simulink model "SimulacionesDT_LUCIA_con_integral"  (R2026b)
settings: Solver=ode15s  StopTime=20
values from neighbouring files (symbols this model uses):
  alpha_Cu = 3.9e-3    (= 0.0039)    [coeficientes.m]
  b_eq = b_m + b_l/(r^2)    (= 2.19444444444e-05)    [coeficientes.m]
  C_ts = 0.818    [coeficientes.m]
  g = 9.80665    [coeficientes.m]
  init_I0 = 0    [coeficientes.m]
  init_Id = 0    [coeficientes.m]
  init_Iq = 0    [coeficientes.m]
  init_theta = 0    [coeficientes.m]
  init_Ts = 20    [coeficientes.m]
  init_w = 0    [coeficientes.m]
  J_eq = J_m + J_l/(r^2)    (= 2.84652777778e-05)    [coeficientes.m]
  k_l = k_l_min + m_l*l_l    (= 0.5)    [coeficientes.m]
  Kd_mov = wn_mov * (2*zeta_mov + 1) * J_eq    (= 0.0569305555556)    [coeficientes.m]
  Ki_mov = wn_mov^3 * J_eq    (= 14574.2222222)    [coeficientes.m]
  Kp_mov = wn_mov^2 * (2*zeta_mov + 1) * J_eq    (= 45.5444444444)    [coeficientes.m]
  L_d = 6.6e-3    (= 0.0066)    [coeficientes.m]
  L_ls = 0.8e-3    (= 0.0008)    [coeficientes.m]
  L_q = 5.8e-3    (= 0.0058)    [coeficientes.m]
  lambda = 0.016    [coeficientes.m]
  Pp = 3    [coeficientes.m]
  r = 120.0    (= 120)    [coeficientes.m]
  R0 = abs(p)*L_ls    [coeficientes.m]
  R_sREF = 1.02    [coeficientes.m]
  R_tsamb = 146.7    [coeficientes.m]
  Rd = abs(p)*L_d    [coeficientes.m]
  Rq = abs(p)*L_q    [coeficientes.m]
  T_sREF = 20    [coeficientes.m]
libraries: eeTransforms x12
(part 2 of 2)

== system SimulacionesDT_LUCIA_con_integral/Sistema con Controlador de Torque Equivalente y sensores ideales1/Modulador de Torque Equivalente/Subsystem ==
  T°s : Inport
  Constant1 : Constant  Value=T_sREF
  Constant2 : Constant
  Gain5 : Gain  Gain=alpha_Cu
  Gain6 : Gain  Gain=R_sREF
  Sum3 : Sum  Inputs=+-|
  Sum4 : Sum  Inputs=|++
  R_s : Outport
  wires:
  Sum3/1 -> Gain5/1
  Sum4/1 -> Gain6/1
  Constant2/1 -> Sum4/2
  Constant1/1 -> Sum3/2
  Gain6/1 -> R_s/1  "R_s"
  Gain5/1 -> Sum4/1
  T°s/1 -> Sum3/1

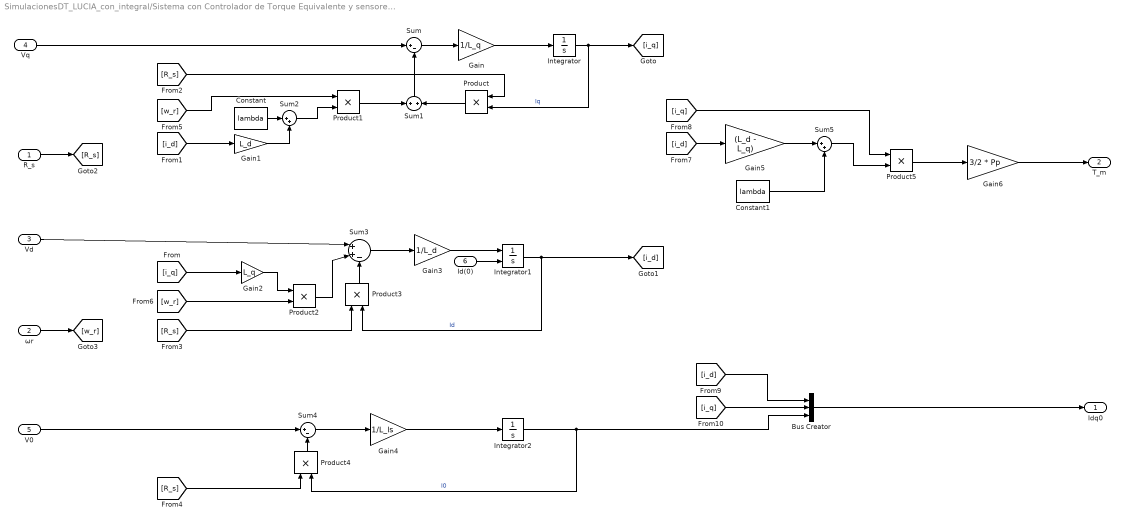
== system SimulacionesDT_LUCIA_con_integral/Sistema con Controlador de Torque Equivalente y sensores ideales1/Planta (Modelo Global No Lineal)/Subsistema Electromagnetico ==
  R_s : Inport
  ωr : Inport  Port=2
  Vd : Inport  Port=3
  Vq : Inport  Port=4
  V0 : Inport  Port=5
  Id(0) : Inport  Port=6
  Bus Creator : BusCreator  Inputs=3
  Constant : Constant  Value=lambda
  Constant1 : Constant  Value=lambda
  Gain : Gain  Gain=1/L_q
  Gain1 : Gain  Gain=L_d
  Gain2 : Gain  Gain=L_q
  Gain3 : Gain  Gain=1/L_d
  Gain4 : Gain  Gain=1/L_ls
  Gain5 : Gain  Gain=(L_d - L_q)
  Gain6 : Gain  Gain=3/2 * Pp
  Integrator : Integrator  InitialCondition=init_Iq
  Integrator1 : Integrator  InitialConditionSource=external  InitialCondition=init_Id
  Integrator2 : Integrator  InitialCondition=init_I0
  Product{,1..5} (6 alike) : Product
  Sum : Sum  Inputs=|+-
  Sum1 : Sum
  Sum2 : Sum  Inputs=|++
  Sum3 : Sum  Inputs=|++-
  Sum4 : Sum  Inputs=|+-
  Sum5 : Sum  Inputs=|++
  Idq0 : Outport
  T_m : Outport  Port=2
  wires:
  [i_q] -> Bus Creator/2
  [i_d] -> Bus Creator/1
  Id(0)/1 -> Integrator1/2
  Bus Creator/1 -> Idq0/1
  [i_q] -> Product5/1
  [i_d] -> Gain5/1
  [w_r] -> Product1/1
  ωr/1 -> [w_r]
  [R_s] -> Product4/1
  [R_s] -> Product3/1
  R_s/1 -> [R_s]
  [i_d] -> Gain1/1
  Gain6/1 -> T_m/1
  Product5/1 -> Gain6/1
  Constant1/1 -> Sum5/2
  Integrator1/1 -> Product3/2, [i_d]  "Id"
  Sum5/1 -> Product5/2
  Gain5/1 -> Sum5/1
  V0/1 -> Sum4/1
  Sum4/1 -> Gain4/1
  Gain4/1 -> Integrator2/1
  Integrator2/1 -> Product4/2, Bus Creator/3  "I0"
  Product4/1 -> Sum4/2
  Vd/1 -> Sum3/1
  Sum3/1 -> Gain3/1
  Gain3/1 -> Integrator1/1
  Product3/1 -> Sum3/3
  Gain/1 -> Integrator/1
  Vq/1 -> Sum/1
  Sum/1 -> Gain/1
  Constant/1 -> Sum2/1
  Sum2/1 -> Product1/2
  Gain1/1 -> Sum2/2
  Product1/1 -> Sum1/1
  Sum1/1 -> Sum/2
  Product/1 -> Sum1/2
  [R_s] -> Product/1
  Integrator/1 -> [i_q], Product/2  "Iq"
  [i_q] -> Gain2/1
  Product2/1 -> Sum3/2
  Gain2/1 -> Product2/1
  [w_r] -> Product2/2

== system SimulacionesDT_LUCIA_con_integral/Sistema con Controlador de Torque Equivalente y sensores ideales1/Planta (Modelo Global No Lineal)/Subsistema Mecanico Equivalente ==
  note: $\theta_m$
  note: $\omega_m$
  note: $\dot{\omega}_m$
  note: $T_{ld}$
  note: $T_m$
  T_m : Inport
  T_ld : Inport  Port=2
  g : Inport  Port=3
  ~θm : Inport  Port=4
  Gain : Gain  Gain=1/r
  Gain1 : Gain  Gain=b_eq
  Gain2 : Gain  Gain=k_l/r
  Gain3 : Gain  Gain=1/J_eq
  Gain4 : Gain  Gain=1/r
  Integrator : Integrator  InitialCondition=init_w
  Integrator1 : Integrator  InitialCondition=init_theta
  Product : Product
  Sin : Trigonometry
  Sum : Sum  Inputs=|+-
  Sum1 : Sum  Inputs=+++
  ωm : Outport
  θm : Outport  Port=2
  wires:
  Integrator1/1 -> Gain4/1, θm/1
  Integrator/1 -> Gain1/1, Integrator1/1, ωm/1
  g/1 -> Product/1
  Product/1 -> Sum1/2
  T_ld/1 -> Gain/1
  Gain4/1 -> Sin/1
  Gain3/1 -> Integrator/1
  Gain1/1 -> Sum1/3
  Sin/1 -> Gain2/1
  Gain/1 -> Sum1/1
  Gain2/1 -> Product/2
  Sum1/1 -> Sum/2
  T_m/1 -> Sum/1
  Sum/1 -> Gain3/1

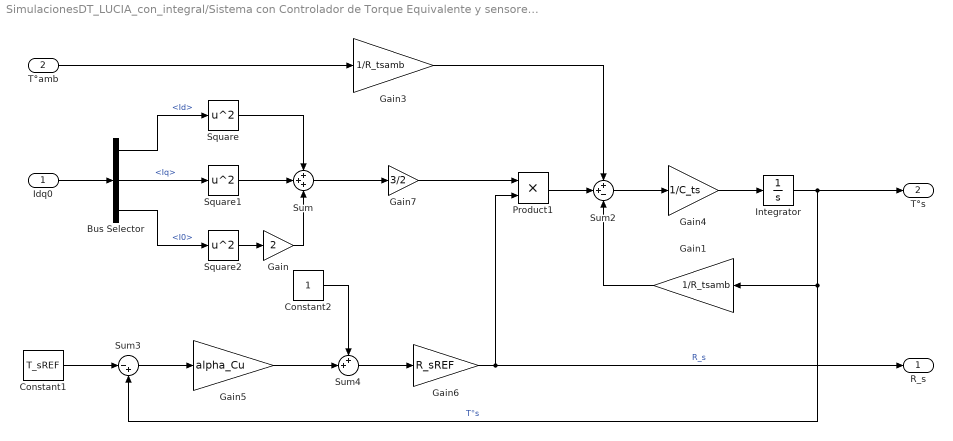
== system SimulacionesDT_LUCIA_con_integral/Sistema con Controlador de Torque Equivalente y sensores ideales1/Planta (Modelo Global No Lineal)/Subsistema Termico ==
  Idq0 : Inport
  T°amb : Inport  Port=2
  Bus Selector : BusSelector  OutputSignals=Id,Iq,I0
  Constant1 : Constant  Value=T_sREF
  Constant2 : Constant
  Gain : Gain  Gain=2
  Gain1 : Gain  Gain=1/R_tsamb
  Gain3 : Gain  Gain=1/R_tsamb
  Gain4 : Gain  Gain=1/C_ts
  Gain5 : Gain  Gain=alpha_Cu
  Gain6 : Gain  Gain=R_sREF
  Gain7 : Gain  Gain=3/2
  Integrator : Integrator  InitialCondition=init_Ts
  Product1 : Product
  Square : Math  Operator=square
  Square1 : Math  Operator=square
  Square2 : Math  Operator=square
  Sum : Sum  Inputs=+++
  Sum2 : Sum  Inputs=++-
  Sum3 : Sum  Inputs=|-+
  Sum4 : Sum  Inputs=++|
  R_s : Outport
  T°s : Outport  Port=2
  wires:
  Bus Selector/3 -> Square2/1  "<I0>"
  Bus Selector/1 -> Square/1  "<Id>"
  Constant2/1 -> Sum4/1
  Idq0/1 -> Bus Selector/1
  Gain3/1 -> Sum2/1
  Gain1/1 -> Sum2/3
  Gain4/1 -> Integrator/1
  Product1/1 -> Sum2/2
  Square/1 -> Sum/1
  Sum2/1 -> Gain4/1
  Square2/1 -> Gain/1
  Sum/1 -> Gain7/1
  T°amb/1 -> Gain3/1
  Sum3/1 -> Gain5/1
  Gain5/1 -> Sum4/2
  Gain/1 -> Sum/3
  Constant1/1 -> Sum3/1
  Sum4/1 -> Gain6/1
  Gain7/1 -> Product1/1
  Gain6/1 -> Product1/2, R_s/1  "R_s"
  Integrator/1 -> T°s/1, Gain1/1, Sum3/2  "T°s"
  Square1/1 -> Sum/2
  Bus Selector/2 -> Square1/1  "<Iq>"

== system SimulacionesDT_LUCIA_con_integral/Sistema con Controlador de Torque Equivalente y sensores ideales1/Planta (Modelo Global No Lineal)/Transformada Directa de Park ==
  Vabc : Inport  OutDataTypeStr=Bus: Vabc
  θm : Inport  Port=2
  Bus Creator : BusCreator  Inputs=3
  Demux : Demux  Outputs=3
  Gain3 : Gain  Gain=Pp
  MATLAB Function2 : MATLAB Function  Commented=on  TreatAsAtomicUnit=on
  Park Transform : eeTransforms/Park Transform  AxisAlignment=Q-axis  PowerInvariant=off
      settings: LibrarySourceBlock=|
      | ee_sl_lib/Mathematical
      | Transforms/Park Transform
  Vdq0 : Outport  OutDataTypeStr=Bus: Vdq0
  wires:
  Gain3/1 -> Park Transform/2
  Demux/1 -> Bus Creator/1  "Vd"
  Demux/3 -> Bus Creator/3  "V0"
  Demux/2 -> Bus Creator/2  "Vq"
  Bus Creator/1 -> Vdq0/1
  θm/1 -> Gain3/1
  Park Transform/1 -> Demux/1  "v_dq0"
  Vabc/1 -> Park Transform/1

== system SimulacionesDT_LUCIA_con_integral/Sistema con Controlador de Torque Equivalente y sensores ideales/Modulador de Torque Equivalente/Lazo de Control de Corrientes Virtuales/Transformada Directa de Park ==
  Iabc : Inport
  θm : Inport  Port=2
  Bus Creator : BusCreator  Inputs=3
  Demux : Demux  Outputs=3
  Gain3 : Gain  Gain=Pp
  Park Transform : eeTransforms/Park Transform  AxisAlignment=Q-axis  PowerInvariant=off
      settings: LibrarySourceBlock=|
      | ee_sl_lib/Mathematical
      | Transforms/Park Transform
  Idq0 : Outport
  wires:
  θm/1 -> Gain3/1
  Iabc/1 -> Park Transform/1
  Bus Creator/1 -> Idq0/1
  Demux/2 -> Bus Creator/2  "Iq"
  Demux/3 -> Bus Creator/3  "I0"
  Demux/1 -> Bus Creator/1  "Id"
  Park Transform/1 -> Demux/1  "Idq0"
  Gain3/1 -> Park Transform/2

== system SimulacionesDT_LUCIA_con_integral/Sistema con Controlador de Torque Equivalente y sensores ideales/Modulador de Torque Equivalente/Modulador de Tensiones Virtuales/Subsystem Reference ==
  θm : Inport
  Vd : Inport  Port=2
  Vq : Inport  Port=3
  V0 : Inport  Port=4
  Bus Creator : BusCreator  Inputs=3
  Bus Creator1 : BusCreator  Inputs=3
  Demux : Demux  Outputs=3
  Gain3 : Gain  Gain=Pp
  Inverse Park Transform : eeTransforms/Inverse Park Transform  AxisAlignment=Q-axis  PowerInvariant=off
      settings: LibrarySourceBlock=|
      | ee_sl_lib/Mathematical
      | Transforms/Inverse
      | Park Transform
  Vdq0 : Outport
  Vabc : Outport  Port=2
  wires:
  Gain3/1 -> Inverse Park Transform/2
  Inverse Park Transform/1 -> Demux/1  "v_abc"
  Demux/1 -> Bus Creator/1  "Va"
  Demux/3 -> Bus Creator/3  "Vc"
  Demux/2 -> Bus Creator/2  "Vb"
  Bus Creator/1 -> Vabc/1
  θm/1 -> Gain3/1
  Vd/1 -> Bus Creator1/1
  Vq/1 -> Bus Creator1/2
  V0/1 -> Bus Creator1/3
  Bus Creator1/1 -> Vdq0/1, Inverse Park Transform/1

== system SimulacionesDT_LUCIA_con_integral/Sistema con Controlador de Torque Equivalente y sensores ideales/Modulador de Torque Equivalente/Modulador de Tensiones Virtuales/Transformada Directa de Park ==
  Iabc : Inport
  θm : Inport  Port=2
  Bus Creator : BusCreator  Inputs=3
  Demux : Demux  Outputs=3
  Gain3 : Gain  Gain=Pp
  Park Transform : eeTransforms/Park Transform  AxisAlignment=Q-axis  PowerInvariant=off
      settings: LibrarySourceBlock=|
      | ee_sl_lib/Mathematical
      | Transforms/Park Transform
  Idq0 : Outport
  wires:
  Gain3/1 -> Park Transform/2
  Park Transform/1 -> Demux/1  "Idq0"
  Demux/1 -> Bus Creator/1  "Id"
  Demux/3 -> Bus Creator/3  "I0"
  Demux/2 -> Bus Creator/2  "Iq"
  Bus Creator/1 -> Idq0/1
  Iabc/1 -> Park Transform/1
  θm/1 -> Gain3/1

== system SimulacionesDT_LUCIA_con_integral/Sistema con Controlador de Torque Equivalente y sensores ideales/Modulador de Torque Equivalente/Modulador y Compensación de Torque/Transformada Directa de Park ==
  θm : Inport
  Iabc : Inport  Port=2
  Bus Creator : BusCreator  Inputs=3
  Demux : Demux  Outputs=3
  Gain3 : Gain  Gain=Pp
  Park Transform : eeTransforms/Park Transform  AxisAlignment=Q-axis  PowerInvariant=off
      settings: LibrarySourceBlock=|
      | ee_sl_lib/Mathematical
      | Transforms/Park Transform
  Idq0 : Outport
  wires:
  θm/1 -> Gain3/1
  Iabc/1 -> Park Transform/1
  Bus Creator/1 -> Idq0/1
  Demux/2 -> Bus Creator/2  "Iq"
  Demux/3 -> Bus Creator/3  "I0"
  Demux/1 -> Bus Creator/1  "Id"
  Park Transform/1 -> Demux/1  "Idq0"
  Gain3/1 -> Park Transform/2

== system SimulacionesDT_LUCIA_con_integral/Sistema con Controlador de Torque Equivalente y sensores ideales1/Modulador de Torque Equivalente/Lazo de Control de Corrientes Virtuales/Transformada Directa de Park ==
  Iabc : Inport
  θm : Inport  Port=2
  Bus Creator : BusCreator  Inputs=3
  Demux : Demux  Outputs=3
  Gain3 : Gain  Gain=Pp
  Park Transform : eeTransforms/Park Transform  AxisAlignment=Q-axis  PowerInvariant=off
      settings: LibrarySourceBlock=|
      | ee_sl_lib/Mathematical
      | Transforms/Park Transform
  Idq0 : Outport
  wires:
  θm/1 -> Gain3/1
  Iabc/1 -> Park Transform/1
  Bus Creator/1 -> Idq0/1
  Demux/2 -> Bus Creator/2  "Iq"
  Demux/3 -> Bus Creator/3  "I0"
  Demux/1 -> Bus Creator/1  "Id"
  Park Transform/1 -> Demux/1  "Idq0"
  Gain3/1 -> Park Transform/2

== system SimulacionesDT_LUCIA_con_integral/Sistema con Controlador de Torque Equivalente y sensores ideales1/Modulador de Torque Equivalente/Modulador de Tensiones Virtuales/Subsystem Reference ==
  θm : Inport
  Vd : Inport  Port=2
  Vq : Inport  Port=3
  V0 : Inport  Port=4
  Bus Creator : BusCreator  Inputs=3
  Bus Creator1 : BusCreator  Inputs=3
  Demux : Demux  Outputs=3
  Gain3 : Gain  Gain=Pp
  Inverse Park Transform : eeTransforms/Inverse Park Transform  AxisAlignment=Q-axis  PowerInvariant=off
      settings: LibrarySourceBlock=|
      | ee_sl_lib/Mathematical
      | Transforms/Inverse
      | Park Transform
  Vdq0 : Outport
  Vabc : Outport  Port=2
  wires:
  Gain3/1 -> Inverse Park Transform/2
  Inverse Park Transform/1 -> Demux/1  "v_abc"
  Demux/1 -> Bus Creator/1  "Va"
  Demux/3 -> Bus Creator/3  "Vc"
  Demux/2 -> Bus Creator/2  "Vb"
  Bus Creator/1 -> Vabc/1
  θm/1 -> Gain3/1
  Vd/1 -> Bus Creator1/1
  Vq/1 -> Bus Creator1/2
  V0/1 -> Bus Creator1/3
  Bus Creator1/1 -> Vdq0/1, Inverse Park Transform/1

== system SimulacionesDT_LUCIA_con_integral/Sistema con Controlador de Torque Equivalente y sensores ideales1/Modulador de Torque Equivalente/Modulador de Tensiones Virtuales/Transformada Directa de Park ==
  Iabc : Inport
  θm : Inport  Port=2
  Bus Creator : BusCreator  Inputs=3
  Demux : Demux  Outputs=3
  Gain3 : Gain  Gain=Pp
  Park Transform : eeTransforms/Park Transform  AxisAlignment=Q-axis  PowerInvariant=off
      settings: LibrarySourceBlock=|
      | ee_sl_lib/Mathematical
      | Transforms/Park Transform
  Idq0 : Outport
  wires:
  Gain3/1 -> Park Transform/2
  Park Transform/1 -> Demux/1  "Idq0"
  Demux/1 -> Bus Creator/1  "Id"
  Demux/3 -> Bus Creator/3  "I0"
  Demux/2 -> Bus Creator/2  "Iq"
  Bus Creator/1 -> Idq0/1
  Iabc/1 -> Park Transform/1
  θm/1 -> Gain3/1

== system SimulacionesDT_LUCIA_con_integral/Sistema con Controlador de Torque Equivalente y sensores ideales1/Modulador de Torque Equivalente/Modulador y Compensación de Torque/Transformada Directa de Park ==
  θm : Inport
  Iabc : Inport  Port=2
  Bus Creator : BusCreator  Inputs=3
  Demux : Demux  Outputs=3
  Gain3 : Gain  Gain=Pp
  Park Transform : eeTransforms/Park Transform  AxisAlignment=Q-axis  PowerInvariant=off
      settings: LibrarySourceBlock=|
      | ee_sl_lib/Mathematical
      | Transforms/Park Transform
  Idq0 : Outport
  wires:
  θm/1 -> Gain3/1
  Iabc/1 -> Park Transform/1
  Bus Creator/1 -> Idq0/1
  Demux/2 -> Bus Creator/2  "Iq"
  Demux/3 -> Bus Creator/3  "I0"
  Demux/1 -> Bus Creator/1  "Id"
  Park Transform/1 -> Demux/1  "Idq0"
  Gain3/1 -> Park Transform/2

== matlab function SimulacionesDT_LUCIA_con_integral/Sistema con Controlador de Torque Equivalente y sensores ideales/Planta (Modelo Global No Lineal)/Transformada Directa de Park/MATLAB Function2 ==
  data: Vabc input; Vdq0 output; theta input
function Vdq0 = TDP_Tension(Vabc, theta)

P = [cos(theta),    cos(theta-2*pi/3),  cos(theta-2*pi/3);...
    sin(theta),     sin(theta-2*pi/3),  sin(theta-2*pi/3);...
    1/2,            1/2,                1/2;];

Vdq0 = 2/3 * P * Vabc;

== matlab function SimulacionesDT_LUCIA_con_integral/Sistema con Controlador de Torque Equivalente y sensores ideales1/Planta (Modelo Global No Lineal)/Transformada Directa de Park/MATLAB Function2 ==
  data: Vabc input; Vdq0 output; theta input
function Vdq0 = TDP_Tension(Vabc, theta)

P = [cos(theta),    cos(theta-2*pi/3),  cos(theta-2*pi/3);...
    sin(theta),     sin(theta-2*pi/3),  sin(theta-2*pi/3);...
    1/2,            1/2,                1/2;];

Vdq0 = 2/3 * P * Vabc;
